simulink model "copia 15_10_26"  (R2026a)
settings: Solver=VariableStepAuto  StopTime=10  RelTol=1e-2  AbsTol=1e-2  EnableMultiTasking=on
values from neighbouring files (symbols this model uses):
  effective_bulkmodulus = 750e6    (= 750000000)    [MARLUP_hydr_params.m]
  m_load = 20    [MARLUP_hydr_params.m]
  p_supply = 160e5    (= 16000000)    [MARLUP_hydr_params.m]
  p_tank = 1.01325e5    (= 101325)    [MARLUP_hydr_params.m]
undefined symbols (not defined in the file or in its folder): cyl, Kd_heave, Kd_pitch, Kd_roll, Ki_heave, Ki_pitch, Ki_roll, Kp_heave, Kp_pitch, Kp_roll, pipe, Tinv, Ts, valve, X, Y, Z
libraries: sm_lib x75, nesl_utility x14, slpidlib x6, simulink x3
(part 4 of 5)

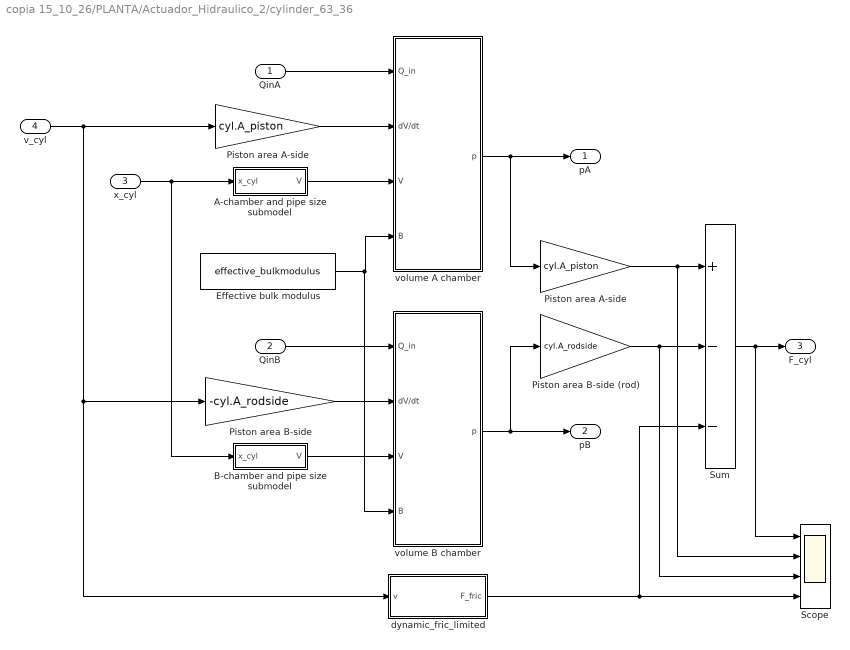
== system copia 15_10_26/PLANTA/Actuador_Hidraulico_2/cylinder_63_36 ==
  QinA : Inport
  QinB : Inport  Port=2
  x_cyl : Inport  Port=3
  v_cyl : Inport  Port=4
  A-chamber and pipe size submodel : Subsystem
  B-chamber and pipe size submodel : Subsystem
  Effective bulk modulus : Constant  Value=effective_bulkmodulus
  Piston area A-side : Gain  Gain=cyl.A_piston
  Piston area B-side (rod) : Gain  Gain=cyl.A_rodside
  Piston area A-side : Gain  Gain=cyl.A_piston
  Piston area B-side : Gain  Gain=-cyl.A_rodside
  Scope : Scope  NumInputPorts=4
      settings: ActiveDisplayYMinimum=-3356.48237  ActiveDisplayYMaximum=15799.75819
  Sum : Sum  Inputs=+--
  dynamic_fric_limited : Subsystem
  volume A chamber : Subsystem
  volume B chamber : Subsystem
  pA : Outport  VectorParamsAs1DForOutWhenUnconnected=off
  pB : Outport  Port=2  VectorParamsAs1DForOutWhenUnconnected=off
  F_cyl : Outport  Port=3  VectorParamsAs1DForOutWhenUnconnected=off
  wires:
  Piston area A-side/1 -> Scope/2, Sum/1
  volume A chamber/1(p) -> pA/1, Piston area A-side/1
  x_cyl/1 -> B-chamber and pipe size submodel/1(x_cyl), A-chamber and pipe size submodel/1(x_cyl)
  v_cyl/1 -> dynamic_fric_limited/1(v), Piston area B-side/1, Piston area A-side/1
  Piston area A-side/1 -> volume A chamber/2(" dV/dt")
  Effective bulk modulus/1 -> volume B chamber/4(" B"), volume A chamber/4(" B")
  Sum/1 -> Scope/1, F_cyl/1
  QinA/1 -> volume A chamber/1(Q_in)
  volume B chamber/1(p) -> pB/1, Piston area B-side (rod)/1
  Piston area B-side (rod)/1 -> Scope/3, Sum/2
  A-chamber and pipe size submodel/1(V) -> volume A chamber/3(" V")
  QinB/1 -> volume B chamber/1(Q_in)
  B-chamber and pipe size submodel/1(V) -> volume B chamber/3(" V")
  Piston area B-side/1 -> volume B chamber/2(" dV/dt")
  dynamic_fric_limited/1(F_fric) -> Sum/3, Scope/4

== system copia 15_10_26/PLANTA/Actuador_Hidraulico_2/gate_load_mass ==
  F_cyl : Inport
  Add : Sum
  Gain : Gain  Gain=1/m_load
  Integrator : Integrator
  Integrator1 : Integrator  InitialCondition=cyl.x_init
  load_fric : Subsystem
  x_cyl : Outport  VectorParamsAs1DForOutWhenUnconnected=off
  v_cyl : Outport  Port=2  VectorParamsAs1DForOutWhenUnconnected=off
  wires:
  Add/1 -> Gain/1
  Gain/1 -> Integrator/1  "accel"
  Integrator/1 -> load_fric/1(v), v_cyl/1, Integrator1/1  "velocity"
  Integrator1/1 -> x_cyl/1  "position"
  F_cyl/1 -> Add/1
  load_fric/1(F_fric_load) -> Add/2

== system copia 15_10_26/PLANTA/Actuador_Hidraulico_3/4_3_directional_valve ==
  pA : Inport
  pB : Inport  Port=2
  u : Inport  Port=3
  Port flows : Subsystem
  Relative opening of flow paths : Subsystem
  Supply pressure : Constant  Value=p_supply
  Tank pressure : Constant  Value=p_tank
  Valve dynamics : Subsystem
  QA : Outport  VectorParamsAs1DForOutWhenUnconnected=off
  QB : Outport  Port=2  VectorParamsAs1DForOutWhenUnconnected=off
  "Q_tank " : Outport  Port=3  VectorParamsAs1DForOutWhenUnconnected=off
  Q_pump : Outport  Port=4  VectorParamsAs1DForOutWhenUnconnected=off
  wires:
  pA/1 -> Port flows/5(pA)
  pB/1 -> Port flows/6(pB)
  Valve dynamics/1(x) -> Relative opening of flow paths/1(x)
  Port flows/3(Q from port T) -> "Q_tank "/1
  Port flows/4(Q from port S) -> Q_pump/1
  Relative opening of flow paths/1(av_SA) -> Port flows/1(av_SA)
  Relative opening of flow paths/2(av_AT) -> Port flows/2(av_AT)
  Relative opening of flow paths/4(av_SB) -> Port flows/4(av_SB)
  u/1 -> Valve dynamics/1(u)
  Port flows/2(Q from port A) -> QA/1
  Port flows/1(Q from port B) -> QB/1
  Supply pressure/1 -> Port flows/7(pS)
  Tank pressure/1 -> Port flows/8(pT)
  Relative opening of flow paths/3(av_BT) -> Port flows/3(av_BT)

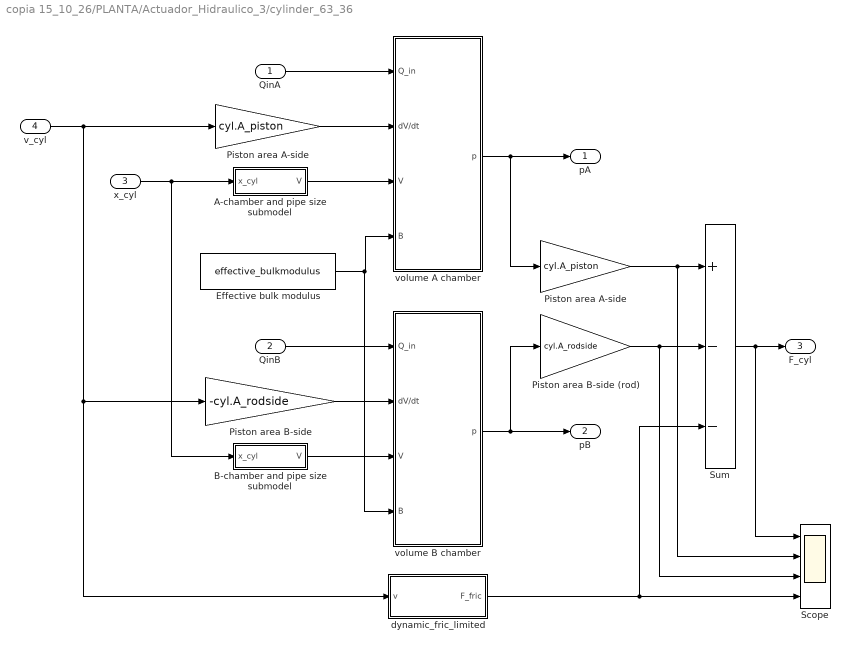
== system copia 15_10_26/PLANTA/Actuador_Hidraulico_3/cylinder_63_36 ==
  QinA : Inport
  QinB : Inport  Port=2
  x_cyl : Inport  Port=3
  v_cyl : Inport  Port=4
  A-chamber and pipe size submodel : Subsystem
  B-chamber and pipe size submodel : Subsystem
  Effective bulk modulus : Constant  Value=effective_bulkmodulus
  Piston area A-side : Gain  Gain=cyl.A_piston
  Piston area B-side (rod) : Gain  Gain=cyl.A_rodside
  Piston area A-side : Gain  Gain=cyl.A_piston
  Piston area B-side : Gain  Gain=-cyl.A_rodside
  Scope : Scope  NumInputPorts=4
      settings: ActiveDisplayYMinimum=-3356.48237  ActiveDisplayYMaximum=15799.75819
  Sum : Sum  Inputs=+--
  dynamic_fric_limited : Subsystem
  volume A chamber : Subsystem
  volume B chamber : Subsystem
  pA : Outport  VectorParamsAs1DForOutWhenUnconnected=off
  pB : Outport  Port=2  VectorParamsAs1DForOutWhenUnconnected=off
  F_cyl : Outport  Port=3  VectorParamsAs1DForOutWhenUnconnected=off
  wires:
  Piston area A-side/1 -> Scope/2, Sum/1
  volume A chamber/1(p) -> pA/1, Piston area A-side/1
  x_cyl/1 -> B-chamber and pipe size submodel/1(x_cyl), A-chamber and pipe size submodel/1(x_cyl)
  v_cyl/1 -> dynamic_fric_limited/1(v), Piston area B-side/1, Piston area A-side/1
  Piston area A-side/1 -> volume A chamber/2(" dV/dt")
  Effective bulk modulus/1 -> volume B chamber/4(" B"), volume A chamber/4(" B")
  Sum/1 -> Scope/1, F_cyl/1
  QinA/1 -> volume A chamber/1(Q_in)
  volume B chamber/1(p) -> pB/1, Piston area B-side (rod)/1
  Piston area B-side (rod)/1 -> Scope/3, Sum/2
  A-chamber and pipe size submodel/1(V) -> volume A chamber/3(" V")
  QinB/1 -> volume B chamber/1(Q_in)
  B-chamber and pipe size submodel/1(V) -> volume B chamber/3(" V")
  Piston area B-side/1 -> volume B chamber/2(" dV/dt")
  dynamic_fric_limited/1(F_fric) -> Sum/3, Scope/4

== system copia 15_10_26/PLANTA/Actuador_Hidraulico_3/gate_load_mass ==
  F_cyl : Inport
  Add : Sum
  Gain : Gain  Gain=1/m_load
  Integrator : Integrator
  Integrator1 : Integrator  InitialCondition=cyl.x_init
  load_fric : Subsystem
  x_cyl : Outport  VectorParamsAs1DForOutWhenUnconnected=off
  v_cyl : Outport  Port=2  VectorParamsAs1DForOutWhenUnconnected=off
  wires:
  Add/1 -> Gain/1
  Gain/1 -> Integrator/1  "accel"
  Integrator/1 -> load_fric/1(v), v_cyl/1, Integrator1/1  "velocity"
  Integrator1/1 -> x_cyl/1  "position"
  F_cyl/1 -> Add/1
  load_fric/1(F_fric_load) -> Add/2

== system copia 15_10_26/PLANTA/Piston 2/Garra 3 ==
  File Solid3 : sm_lib/Body Elements/File Solid  ExtGeomFileName=rotate.SLDPRT  UnitType=FromFile  ExtGeomFileUnits=m  StepReaderType=HEX  ExportConvexHullGeometry=off  InertiaType=CalculateFromGeometry  BasedOnType=DensityFromFile  Density=1000  DensityUnits=kg/m^3  Mass=1  MassUnits=kg  CenterOfMass=[0 0 0]  CenterOfMassUnits=m  MomentsOfInertia=[1 1 1]  MomentsOfInertiaUnits=kg*m^2  ProductsOfInertia=[0 0 0]  ProductsOfInertiaUnits=kg*m^2  GraphicType=FromGeometry  MarkerShape=Sphere  MarkerSize=10  GraphicVisPropType=SimpleVisualProperties  GraphicDiffuseColor=[0.5 0.5 0.5]  GraphicOpacity=1  GraphicSpecularColor=[0.5 0.5 0.5 1.0]  GraphicAmbientColor=[0.15 0.15 0.15 1.0]  GraphicEmissiveColor=[0.0 0.0 0.0 1.0]  GraphicShininess=75  DoExposeReferenceFrame=off  SerializedFrames=<Frames><Frame><Id>Frame2</Id><Value><Name>F2</Name><Origin><Source>GeometricFeature</Source><FeatureName>circular curve 40</FeatureName></Origin><PrimaryAxis><DefinedDirection>+Z</DefinedDirection><Source>ReferenceFrame</Source><SourceDirection>+Z</SourceDirection><FeatureName></FeatureName></PrimaryAxis><SecondaryAxis><DefinedDirection>+X</DefinedDirection><Source>ReferenceFrame</Source><SourceDirection>+X</SourceDirection><FeatureName></FeatureName></SecondaryAxis></Value></Frame><Frame><Id>Frame3</Id><Value><Name>F3-1</Name><Origin><Source>GeometricFeature</Source><FeatureName>planar surface 7</FeatureName></Origin><PrimaryAxis><DefinedDirection>+Z</DefinedDirection><Source>ReferenceFrame</Source><SourceDirection>+Z</SourceDirection><FeatureName></FeatureName></PrimaryAxis><SecondaryAxis><DefinedDirection>+X</DefinedDirection><Source>ReferenceFrame</Source><SourceDirection>+X</SourceDirection><FeatureName></FeatureName></SecondaryAxis></Value></Frame></Frames>
  Join block 1 : sm_lib/Body Elements/File Solid  ExtGeomFileName=joint_block.SLDPRT  UnitType=FromFile  ExtGeomFileUnits=m  StepReaderType=HEX  ExportConvexHullGeometry=off  InertiaType=CalculateFromGeometry  BasedOnType=DensityFromFile  Density=1000  DensityUnits=kg/m^3  Mass=1  MassUnits=kg  CenterOfMass=[0 0 0]  CenterOfMassUnits=m  MomentsOfInertia=[1 1 1]  MomentsOfInertiaUnits=kg*m^2  ProductsOfInertia=[0 0 0]  ProductsOfInertiaUnits=kg*m^2  GraphicType=FromGeometry  MarkerShape=Sphere  MarkerSize=10  GraphicVisPropType=SimpleVisualProperties  GraphicDiffuseColor=[0.5 0.5 0.5]  GraphicOpacity=1  GraphicSpecularColor=[0.5 0.5 0.5 1.0]  GraphicAmbientColor=[0.15 0.15 0.15 1.0]  GraphicEmissiveColor=[0.0 0.0 0.0 1.0]  GraphicShininess=75  DoExposeReferenceFrame=off  SerializedFrames=<Frames><Frame><Id>Frame1</Id><Value><Name>F1</Name><Origin><Source>GeometricFeature</Source><FeatureName>circular curve 40</FeatureName></Origin><PrimaryAxis><DefinedDirection>+Z</DefinedDirection><Source>ReferenceFrame</Source><SourceDirection>+X</SourceDirection><FeatureName></FeatureName></PrimaryAxis><SecondaryAxis><DefinedDirection>-X</DefinedDirection><Source>ReferenceFrame</Source><SourceDirection>+Z</SourceDirection><FeatureName></FeatureName></SecondaryAxis></Value></Frame><Frame><Id>Frame2</Id><Value><Name>F2</Name><Origin><Source>GeometricFeature</Source><FeatureName>circular curve 35</FeatureName></Origin><PrimaryAxis><DefinedDirection>+Z</DefinedDirection><Source>ReferenceFrame</Source><SourceDirection>+Z</SourceDirection><FeatureName></FeatureName></PrimaryAxis><SecondaryAxis><DefinedDirection>+X</DefinedDirection><Source>ReferenceFrame</Source><SourceDirection>+X</SourceDirection><FeatureName></FeatureName></SecondaryAxis></Value></Frame></Frames>
  Revolute Joint : sm_lib/Joints/Revolute Joint  JointMode=Normal  CompositeWrenchDir=FollowerOnBase  CompositeWrenchFrame=BaseFrame  SenseConstraintForce=off  SenseConstraintTorque=off  SenseTotalForce=off  SenseTotalTorque=off  PositionTargetSpecify=off  PositionTargetPriority=High  PositionTargetValue=-43.6009  PositionTargetValueUnits=deg  VelocityTargetSpecify=off  VelocityTargetPriority=High  VelocityTargetValue=0  VelocityTargetValueUnits=deg/s  EquilibriumPosition=0  EquilibriumPositionUnits=deg  SpringStiffness=0  SpringStiffnessUnits=N*m/deg  DampingCoefficient=1.5e-4  DampingCoefficientUnits=N*m/(deg/s)  LowerLimitSpecify=off  LowerLimitBound=-90  LowerLimitBoundUnits=deg  LowerLimitStiffness=1e4  LowerLimitStiffnessUnits=N*m/deg  LowerLimitDamping=10  LowerLimitDampingUnits=N*m/(deg/s)  LowerLimitTransitionRegionWidth=0.1  LowerLimitTransitionRegionWidthUnits=deg  UpperLimitSpecify=off  UpperLimitBound=90  UpperLimitBoundUnits=deg  UpperLimitStiffness=1e4  UpperLimitStiffnessUnits=N*m/deg  UpperLimitDamping=10  UpperLimitDampingUnits=N*m/(deg/s)  UpperLimitTransitionRegionWidth=0.1  UpperLimitTransitionRegionWidthUnits=deg  TorqueActuationMode=NoTorque  MotionActuationMode=ComputedMotion  SensePosition=off  SenseVelocity=off  SenseAcceleration=off  SenseTorqueForce=off  SenseLowerLimitTorqueForce=off  SenseUpperLimitTorqueForce=off
  Rigid Transform3 : sm_lib/Frames and Transforms/Rigid Transform  RotationMethod=RotationSequence  FollAlignAxisA=+X  BaseAlignAxisA=+Y  FollAlignAxisB=+Y  BaseAlignAxisB=+Z  RotationStandardAxis=+Y  RotationAngle=-30  RotationAngleUnits=deg  RotationArbitraryAxis=[0 0 1]  RotationSequenceAxes=FollowerAxes  RotationSequence=XYZ  RotationSequenceAngles=[2 -180 180]  RotationSequenceAnglesUnits=deg  RotationMatrix=[1 0 0;0 1 0;0 0 1]  Quaternion=[1 0 0 0]  TranslationMethod=None  TranslationCartesianOffset=[0 0 0]  TranslationCartesianOffsetUnits=m  TranslationStandardAxis=+Z  TranslationStandardOffset=0  TranslationStandardOffsetUnits=m  TranslationROffset=0  TranslationROffsetUnits=m  TranslationThetaOffset=0  TranslationThetaOffsetUnits=deg  TranslationZOffset=0  TranslationZOffsetUnits=m
  Rotate 1 : sm_lib/Body Elements/File Solid  ExtGeomFileName=rotate2.SLDPRT  UnitType=FromFile  ExtGeomFileUnits=m  StepReaderType=HEX  ExportConvexHullGeometry=off  InertiaType=CalculateFromGeometry  BasedOnType=DensityFromFile  Density=1000  DensityUnits=kg/m^3  Mass=1  MassUnits=kg  CenterOfMass=[0 0 0]  CenterOfMassUnits=m  MomentsOfInertia=[1 1 1]  MomentsOfInertiaUnits=kg*m^2  ProductsOfInertia=[0 0 0]  ProductsOfInertiaUnits=kg*m^2  GraphicType=FromGeometry  MarkerShape=Sphere  MarkerSize=10  GraphicVisPropType=SimpleVisualProperties  GraphicDiffuseColor=[0.5 0.5 0.5]  GraphicOpacity=1  GraphicSpecularColor=[0.5 0.5 0.5 1.0]  GraphicAmbientColor=[0.15 0.15 0.15 1.0]  GraphicEmissiveColor=[0.0 0.0 0.0 1.0]  GraphicShininess=75  DoExposeReferenceFrame=off  SerializedFrames=<Frames><Frame><Id>Frame1</Id><Value><Name>F1</Name><Origin><Source>GeometricFeature</Source><FeatureName>circular curve 36</FeatureName></Origin><PrimaryAxis><DefinedDirection>+Y</DefinedDirection><Source>ReferenceFrame</Source><SourceDirection>+Z</SourceDirection><FeatureName></FeatureName></PrimaryAxis><SecondaryAxis><DefinedDirection>+X</DefinedDirection><Source>ReferenceFrame</Source><SourceDirection>+X</SourceDirection><FeatureName></FeatureName></SecondaryAxis></Value></Frame><Frame><Id>Frame2</Id><Value><Name>F2</Name><Origin><Source>GeometricFeature</Source><FeatureName>circular curve 43</FeatureName></Origin><PrimaryAxis><DefinedDirection>+Z</DefinedDirection><Source>ReferenceFrame</Source><SourceDirection>+X</SourceDirection><FeatureName></FeatureName></PrimaryAxis><SecondaryAxis><DefinedDirection>-X</DefinedDirection><Source>ReferenceFrame</Source><SourceDirection>+Z</SourceDirection><FeatureName></FeatureName></SecondaryAxis></Value></Frame></Frames>
  Conn1 : PMIOPort  Side=Left
  Conn2 : PMIOPort  Port=2  Side=Right
  measure_up : PMIOPort  Port=3  Side=Right
  measure_z : PMIOPort  Port=4  Side=Left
  connections:
  Rigid Transform3/LConn1 -- measure_up/RConn1 -- Join block 1/RConn1
  Rotate 1/LConn1 -- Conn1/RConn1
  Conn2/RConn1 -- File Solid3/RConn1
  Rotate 1/RConn1 -- Revolute Joint/LConn1
  Join block 1/LConn1 -- measure_z/RConn1 -- Revolute Joint/RConn1
  File Solid3/LConn1 -- Rigid Transform3/RConn1

== system copia 15_10_26/PLANTA/Piston1/Garra 1 ==
  File Solid1 : sm_lib/Body Elements/File Solid  ExtGeomFileName=rotate.SLDPRT  UnitType=FromFile  ExtGeomFileUnits=m  StepReaderType=HEX  ExportConvexHullGeometry=off  InertiaType=CalculateFromGeometry  BasedOnType=DensityFromFile  Density=1000  DensityUnits=kg/m^3  Mass=1  MassUnits=kg  CenterOfMass=[0 0 0]  CenterOfMassUnits=m  MomentsOfInertia=[1 1 1]  MomentsOfInertiaUnits=kg*m^2  ProductsOfInertia=[0 0 0]  ProductsOfInertiaUnits=kg*m^2  GraphicType=FromGeometry  MarkerShape=Sphere  MarkerSize=10  GraphicVisPropType=SimpleVisualProperties  GraphicDiffuseColor=[0.5 0.5 0.5]  GraphicOpacity=1  GraphicSpecularColor=[0.5 0.5 0.5 1.0]  GraphicAmbientColor=[0.15 0.15 0.15 1.0]  GraphicEmissiveColor=[0.0 0.0 0.0 1.0]  GraphicShininess=75  DoExposeReferenceFrame=off  SerializedFrames=<Frames><Frame><Id>Frame2</Id><Value><Name>F2</Name><Origin><Source>GeometricFeature</Source><FeatureName>circular curve 40</FeatureName></Origin><PrimaryAxis><DefinedDirection>+Z</DefinedDirection><Source>ReferenceFrame</Source><SourceDirection>+Z</SourceDirection><FeatureName></FeatureName></PrimaryAxis><SecondaryAxis><DefinedDirection>+X</DefinedDirection><Source>ReferenceFrame</Source><SourceDirection>+X</SourceDirection><FeatureName></FeatureName></SecondaryAxis></Value></Frame><Frame><Id>Frame3</Id><Value><Name>F3-1</Name><Origin><Source>GeometricFeature</Source><FeatureName>planar surface 7</FeatureName></Origin><PrimaryAxis><DefinedDirection>+Z</DefinedDirection><Source>ReferenceFrame</Source><SourceDirection>+Z</SourceDirection><FeatureName></FeatureName></PrimaryAxis><SecondaryAxis><DefinedDirection>+X</DefinedDirection><Source>ReferenceFrame</Source><SourceDirection>+X</SourceDirection><FeatureName></FeatureName></SecondaryAxis></Value></Frame></Frames>
  Join block 2 : sm_lib/Body Elements/File Solid  ExtGeomFileName=joint_block.SLDPRT  UnitType=FromFile  ExtGeomFileUnits=m  StepReaderType=HEX  ExportConvexHullGeometry=off  InertiaType=CalculateFromGeometry  BasedOnType=DensityFromFile  Density=1000  DensityUnits=kg/m^3  Mass=1  MassUnits=kg  CenterOfMass=[0 0 0]  CenterOfMassUnits=m  MomentsOfInertia=[1 1 1]  MomentsOfInertiaUnits=kg*m^2  ProductsOfInertia=[0 0 0]  ProductsOfInertiaUnits=kg*m^2  GraphicType=FromGeometry  MarkerShape=Sphere  MarkerSize=10  GraphicVisPropType=SimpleVisualProperties  GraphicDiffuseColor=[0.5 0.5 0.5]  GraphicOpacity=1  GraphicSpecularColor=[0.5 0.5 0.5 1.0]  GraphicAmbientColor=[0.15 0.15 0.15 1.0]  GraphicEmissiveColor=[0.0 0.0 0.0 1.0]  GraphicShininess=75  DoExposeReferenceFrame=off  SerializedFrames=<Frames><Frame><Id>Frame1</Id><Value><Name>F1</Name><Origin><Source>GeometricFeature</Source><FeatureName>circular curve 40</FeatureName></Origin><PrimaryAxis><DefinedDirection>+Z</DefinedDirection><Source>ReferenceFrame</Source><SourceDirection>+X</SourceDirection><FeatureName></FeatureName></PrimaryAxis><SecondaryAxis><DefinedDirection>-X</DefinedDirection><Source>ReferenceFrame</Source><SourceDirection>+Z</SourceDirection><FeatureName></FeatureName></SecondaryAxis></Value></Frame><Frame><Id>Frame2</Id><Value><Name>F2</Name><Origin><Source>GeometricFeature</Source><FeatureName>circular curve 35</FeatureName></Origin><PrimaryAxis><DefinedDirection>+Z</DefinedDirection><Source>ReferenceFrame</Source><SourceDirection>+Z</SourceDirection><FeatureName></FeatureName></PrimaryAxis><SecondaryAxis><DefinedDirection>+X</DefinedDirection><Source>ReferenceFrame</Source><SourceDirection>+X</SourceDirection><FeatureName></FeatureName></SecondaryAxis></Value></Frame></Frames>
  Revolute Joint : sm_lib/Joints/Revolute Joint  JointMode=Normal  CompositeWrenchDir=FollowerOnBase  CompositeWrenchFrame=BaseFrame  SenseConstraintForce=off  SenseConstraintTorque=off  SenseTotalForce=off  SenseTotalTorque=off  PositionTargetSpecify=off  PositionTargetPriority=High  PositionTargetValue=-45.85  PositionTargetValueUnits=deg  VelocityTargetSpecify=off  VelocityTargetPriority=High  VelocityTargetValue=0  VelocityTargetValueUnits=deg/s  EquilibriumPosition=0  EquilibriumPositionUnits=deg  SpringStiffness=0  SpringStiffnessUnits=N*m/deg  DampingCoefficient=1.5e-4  DampingCoefficientUnits=N*m/(deg/s)  LowerLimitSpecify=off  LowerLimitBound=-90  LowerLimitBoundUnits=deg  LowerLimitStiffness=1e4  LowerLimitStiffnessUnits=N*m/deg  LowerLimitDamping=10  LowerLimitDampingUnits=N*m/(deg/s)  LowerLimitTransitionRegionWidth=0.1  LowerLimitTransitionRegionWidthUnits=deg  UpperLimitSpecify=off  UpperLimitBound=90  UpperLimitBoundUnits=deg  UpperLimitStiffness=1e4  UpperLimitStiffnessUnits=N*m/deg  UpperLimitDamping=10  UpperLimitDampingUnits=N*m/(deg/s)  UpperLimitTransitionRegionWidth=0.1  UpperLimitTransitionRegionWidthUnits=deg  TorqueActuationMode=NoTorque  MotionActuationMode=ComputedMotion  SensePosition=off  SenseVelocity=off  SenseAcceleration=off  SenseTorqueForce=off  SenseLowerLimitTorqueForce=off  SenseUpperLimitTorqueForce=off
  Rigid Transform3 : sm_lib/Frames and Transforms/Rigid Transform  RotationMethod=RotationSequence  FollAlignAxisA=+X  BaseAlignAxisA=+Y  FollAlignAxisB=+Y  BaseAlignAxisB=+Z  RotationStandardAxis=+Y  RotationAngle=-30  RotationAngleUnits=deg  RotationArbitraryAxis=[0 0 1]  RotationSequenceAxes=FollowerAxes  RotationSequence=XYZ  RotationSequenceAngles=[2 -180 180]  RotationSequenceAnglesUnits=deg  RotationMatrix=[1 0 0;0 1 0;0 0 1]  Quaternion=[1 0 0 0]  TranslationMethod=None  TranslationCartesianOffset=[0 0 0]  TranslationCartesianOffsetUnits=m  TranslationStandardAxis=+Z  TranslationStandardOffset=0  TranslationStandardOffsetUnits=m  TranslationROffset=0  TranslationROffsetUnits=m  TranslationThetaOffset=0  TranslationThetaOffsetUnits=deg  TranslationZOffset=0  TranslationZOffsetUnits=m
  Rotate 2 : sm_lib/Body Elements/File Solid  ExtGeomFileName=rotate2.SLDPRT  UnitType=FromFile  ExtGeomFileUnits=m  StepReaderType=HEX  ExportConvexHullGeometry=off  InertiaType=CalculateFromGeometry  BasedOnType=DensityFromFile  Density=1000  DensityUnits=kg/m^3  Mass=1  MassUnits=kg  CenterOfMass=[0 0 0]  CenterOfMassUnits=m  MomentsOfInertia=[1 1 1]  MomentsOfInertiaUnits=kg*m^2  ProductsOfInertia=[0 0 0]  ProductsOfInertiaUnits=kg*m^2  GraphicType=FromGeometry  MarkerShape=Sphere  MarkerSize=10  GraphicVisPropType=SimpleVisualProperties  GraphicDiffuseColor=[0.5 0.5 0.5]  GraphicOpacity=1  GraphicSpecularColor=[0.5 0.5 0.5 1.0]  GraphicAmbientColor=[0.15 0.15 0.15 1.0]  GraphicEmissiveColor=[0.0 0.0 0.0 1.0]  GraphicShininess=75  DoExposeReferenceFrame=off  SerializedFrames=<Frames><Frame><Id>Frame1</Id><Value><Name>F1</Name><Origin><Source>GeometricFeature</Source><FeatureName>circular curve 36</FeatureName></Origin><PrimaryAxis><DefinedDirection>+Y</DefinedDirection><Source>ReferenceFrame</Source><SourceDirection>+Z</SourceDirection><FeatureName></FeatureName></PrimaryAxis><SecondaryAxis><DefinedDirection>+X</DefinedDirection><Source>ReferenceFrame</Source><SourceDirection>+X</SourceDirection><FeatureName></FeatureName></SecondaryAxis></Value></Frame><Frame><Id>Frame2</Id><Value><Name>F2</Name><Origin><Source>GeometricFeature</Source><FeatureName>circular curve 43</FeatureName></Origin><PrimaryAxis><DefinedDirection>+Z</DefinedDirection><Source>ReferenceFrame</Source><SourceDirection>+X</SourceDirection><FeatureName></FeatureName></PrimaryAxis><SecondaryAxis><DefinedDirection>-X</DefinedDirection><Source>ReferenceFrame</Source><SourceDirection>+Z</SourceDirection><FeatureName></FeatureName></SecondaryAxis></Value></Frame></Frames>
  Conn1 : PMIOPort  Side=Left
  Conn2 : PMIOPort  Port=2  Side=Right
  connections:
  Rotate 2/LConn1 -- Conn1/RConn1
  File Solid1/RConn1 -- Conn2/RConn1
  Rigid Transform3/RConn1 -- File Solid1/LConn1
  Rotate 2/RConn1 -- Revolute Joint/LConn1
  Revolute Joint/RConn1 -- Join block 2/LConn1
  Join block 2/RConn1 -- Rigid Transform3/LConn1

== system copia 15_10_26/PLANTA/Piston3/Garra 3 ==
  File Solid3 : sm_lib/Body Elements/File Solid  ExtGeomFileName=rotate.SLDPRT  UnitType=FromFile  ExtGeomFileUnits=m  StepReaderType=HEX  ExportConvexHullGeometry=off  InertiaType=CalculateFromGeometry  BasedOnType=DensityFromFile  Density=1000  DensityUnits=kg/m^3  Mass=1  MassUnits=kg  CenterOfMass=[0 0 0]  CenterOfMassUnits=m  MomentsOfInertia=[1 1 1]  MomentsOfInertiaUnits=kg*m^2  ProductsOfInertia=[0 0 0]  ProductsOfInertiaUnits=kg*m^2  GraphicType=FromGeometry  MarkerShape=Sphere  MarkerSize=10  GraphicVisPropType=SimpleVisualProperties  GraphicDiffuseColor=[0.5 0.5 0.5]  GraphicOpacity=1  GraphicSpecularColor=[0.5 0.5 0.5 1.0]  GraphicAmbientColor=[0.15 0.15 0.15 1.0]  GraphicEmissiveColor=[0.0 0.0 0.0 1.0]  GraphicShininess=75  DoExposeReferenceFrame=off  SerializedFrames=<Frames><Frame><Id>Frame1</Id><Value><Name>F1</Name><Origin><Source>GeometricFeature</Source><FeatureName>circular curve 16</FeatureName></Origin><PrimaryAxis><DefinedDirection>+Z</DefinedDirection><Source>ReferenceFrame</Source><SourceDirection>+Z</SourceDirection><FeatureName></FeatureName></PrimaryAxis><SecondaryAxis><DefinedDirection>+X</DefinedDirection><Source>ReferenceFrame</Source><SourceDirection>+X</SourceDirection><FeatureName></FeatureName></SecondaryAxis></Value></Frame><Frame><Id>Frame2</Id><Value><Name>F2</Name><Origin><Source>GeometricFeature</Source><FeatureName>circular curve 40</FeatureName></Origin><PrimaryAxis><DefinedDirection>+Z</DefinedDirection><Source>ReferenceFrame</Source><SourceDirection>+Z</SourceDirection><FeatureName></FeatureName></PrimaryAxis><SecondaryAxis><DefinedDirection>+X</DefinedDirection><Source>ReferenceFrame</Source><SourceDirection>+X</SourceDirection><FeatureName></FeatureName></SecondaryAxis></Value></Frame><Frame><Id>Frame3</Id><Value><Name>F3-1</Name><Origin><Source>GeometricFeature</Source><FeatureName>planar surface 7</FeatureName></Origin><PrimaryAxis><DefinedDirection>+Z</DefinedDirection><Source>ReferenceFrame</Source><SourceDirection>+Z</SourceDirection><FeatureName></FeatureName></PrimaryAxis><SecondaryAxis><DefinedDirection>+X</DefinedDirection><Source>ReferenceFrame</Source><SourceDirection>+X</SourceDirection><FeatureName></FeatureName></SecondaryAxis></Value></Frame></Frames>
  Join block 1 : sm_lib/Body Elements/File Solid  ExtGeomFileName=joint_block.SLDPRT  UnitType=FromFile  ExtGeomFileUnits=m  StepReaderType=HEX  ExportConvexHullGeometry=off  InertiaType=CalculateFromGeometry  BasedOnType=DensityFromFile  Density=1000  DensityUnits=kg/m^3  Mass=1  MassUnits=kg  CenterOfMass=[0 0 0]  CenterOfMassUnits=m  MomentsOfInertia=[1 1 1]  MomentsOfInertiaUnits=kg*m^2  ProductsOfInertia=[0 0 0]  ProductsOfInertiaUnits=kg*m^2  GraphicType=FromGeometry  MarkerShape=Sphere  MarkerSize=10  GraphicVisPropType=SimpleVisualProperties  GraphicDiffuseColor=[0.5 0.5 0.5]  GraphicOpacity=1  GraphicSpecularColor=[0.5 0.5 0.5 1.0]  GraphicAmbientColor=[0.15 0.15 0.15 1.0]  GraphicEmissiveColor=[0.0 0.0 0.0 1.0]  GraphicShininess=75  DoExposeReferenceFrame=off  SerializedFrames=<Frames><Frame><Id>Frame1</Id><Value><Name>F1</Name><Origin><Source>GeometricFeature</Source><FeatureName>circular curve 40</FeatureName></Origin><PrimaryAxis><DefinedDirection>+Z</DefinedDirection><Source>ReferenceFrame</Source><SourceDirection>+X</SourceDirection><FeatureName></FeatureName></PrimaryAxis><SecondaryAxis><DefinedDirection>-X</DefinedDirection><Source>ReferenceFrame</Source><SourceDirection>+Z</SourceDirection><FeatureName></FeatureName></SecondaryAxis></Value></Frame><Frame><Id>Frame2</Id><Value><Name>F2</Name><Origin><Source>GeometricFeature</Source><FeatureName>circular curve 35</FeatureName></Origin><PrimaryAxis><DefinedDirection>+Z</DefinedDirection><Source>ReferenceFrame</Source><SourceDirection>+Z</SourceDirection><FeatureName></FeatureName></PrimaryAxis><SecondaryAxis><DefinedDirection>+X</DefinedDirection><Source>ReferenceFrame</Source><SourceDirection>+X</SourceDirection><FeatureName></FeatureName></SecondaryAxis></Value></Frame></Frames>
  Revolute Joint : sm_lib/Joints/Revolute Joint  JointMode=Normal  CompositeWrenchDir=FollowerOnBase  CompositeWrenchFrame=BaseFrame  SenseConstraintForce=off  SenseConstraintTorque=off  SenseTotalForce=off  SenseTotalTorque=off  PositionTargetSpecify=off  PositionTargetPriority=High  PositionTargetValue=-43.492  PositionTargetValueUnits=deg  VelocityTargetSpecify=off  VelocityTargetPriority=High  VelocityTargetValue=0  VelocityTargetValueUnits=deg/s  EquilibriumPosition=0  EquilibriumPositionUnits=deg  SpringStiffness=0  SpringStiffnessUnits=N*m/deg  DampingCoefficient=1.5e-4  DampingCoefficientUnits=N*m/(deg/s)  LowerLimitSpecify=off  LowerLimitBound=-90  LowerLimitBoundUnits=deg  LowerLimitStiffness=1e4  LowerLimitStiffnessUnits=N*m/deg  LowerLimitDamping=10  LowerLimitDampingUnits=N*m/(deg/s)  LowerLimitTransitionRegionWidth=0.1  LowerLimitTransitionRegionWidthUnits=deg  UpperLimitSpecify=off  UpperLimitBound=90  UpperLimitBoundUnits=deg  UpperLimitStiffness=1e4  UpperLimitStiffnessUnits=N*m/deg  UpperLimitDamping=10  UpperLimitDampingUnits=N*m/(deg/s)  UpperLimitTransitionRegionWidth=0.1  UpperLimitTransitionRegionWidthUnits=deg  TorqueActuationMode=NoTorque  MotionActuationMode=ComputedMotion  SensePosition=off  SenseVelocity=off  SenseAcceleration=off  SenseTorqueForce=off  SenseLowerLimitTorqueForce=off  SenseUpperLimitTorqueForce=off
  Rigid Transform3 : sm_lib/Frames and Transforms/Rigid Transform  RotationMethod=RotationSequence  FollAlignAxisA=+X  BaseAlignAxisA=+Y  FollAlignAxisB=+Y  BaseAlignAxisB=+Z  RotationStandardAxis=+Y  RotationAngle=-30  RotationAngleUnits=deg  RotationArbitraryAxis=[0 0 1]  RotationSequenceAxes=FollowerAxes  RotationSequence=XYZ  RotationSequenceAngles=[2 -180 180]  RotationSequenceAnglesUnits=deg  RotationMatrix=[1 0 0;0 1 0;0 0 1]  Quaternion=[1 0 0 0]  TranslationMethod=None  TranslationCartesianOffset=[0 0 0]  TranslationCartesianOffsetUnits=m  TranslationStandardAxis=+Z  TranslationStandardOffset=0  TranslationStandardOffsetUnits=m  TranslationROffset=0  TranslationROffsetUnits=m  TranslationThetaOffset=0  TranslationThetaOffsetUnits=deg  TranslationZOffset=0  TranslationZOffsetUnits=m
  Rotate 1 : sm_lib/Body Elements/File Solid  ExtGeomFileName=rotate2.SLDPRT  UnitType=FromFile  ExtGeomFileUnits=m  StepReaderType=HEX  ExportConvexHullGeometry=off  InertiaType=CalculateFromGeometry  BasedOnType=DensityFromFile  Density=1000  DensityUnits=kg/m^3  Mass=1  MassUnits=kg  CenterOfMass=[0 0 0]  CenterOfMassUnits=m  MomentsOfInertia=[1 1 1]  MomentsOfInertiaUnits=kg*m^2  ProductsOfInertia=[0 0 0]  ProductsOfInertiaUnits=kg*m^2  GraphicType=FromGeometry  MarkerShape=Sphere  MarkerSize=10  GraphicVisPropType=SimpleVisualProperties  GraphicDiffuseColor=[0.5 0.5 0.5]  GraphicOpacity=1  GraphicSpecularColor=[0.5 0.5 0.5 1.0]  GraphicAmbientColor=[0.15 0.15 0.15 1.0]  GraphicEmissiveColor=[0.0 0.0 0.0 1.0]  GraphicShininess=75  DoExposeReferenceFrame=off  SerializedFrames=<Frames><Frame><Id>Frame1</Id><Value><Name>F1</Name><Origin><Source>GeometricFeature</Source><FeatureName>circular curve 36</FeatureName></Origin><PrimaryAxis><DefinedDirection>+Y</DefinedDirection><Source>ReferenceFrame</Source><SourceDirection>+Z</SourceDirection><FeatureName></FeatureName></PrimaryAxis><SecondaryAxis><DefinedDirection>+X</DefinedDirection><Source>ReferenceFrame</Source><SourceDirection>+X</SourceDirection><FeatureName></FeatureName></SecondaryAxis></Value></Frame><Frame><Id>Frame2</Id><Value><Name>F2</Name><Origin><Source>GeometricFeature</Source><FeatureName>circular curve 43</FeatureName></Origin><PrimaryAxis><DefinedDirection>+Z</DefinedDirection><Source>ReferenceFrame</Source><SourceDirection>+X</SourceDirection><FeatureName></FeatureName></PrimaryAxis><SecondaryAxis><DefinedDirection>-X</DefinedDirection><Source>ReferenceFrame</Source><SourceDirection>+Z</SourceDirection><FeatureName></FeatureName></SecondaryAxis></Value></Frame></Frames>
  Conn1 : PMIOPort  Side=Left
  Conn2 : PMIOPort  Port=2  Side=Right
  connections:
  Join block 1/RConn1 -- Rigid Transform3/LConn1
  Rigid Transform3/RConn1 -- File Solid3/RConn1
  Rotate 1/LConn1 -- Conn1/RConn1
  File Solid3/LConn2 -- Conn2/RConn1
  Rotate 1/RConn1 -- Revolute Joint/LConn1
  Join block 1/LConn1 -- Revolute Joint/RConn1

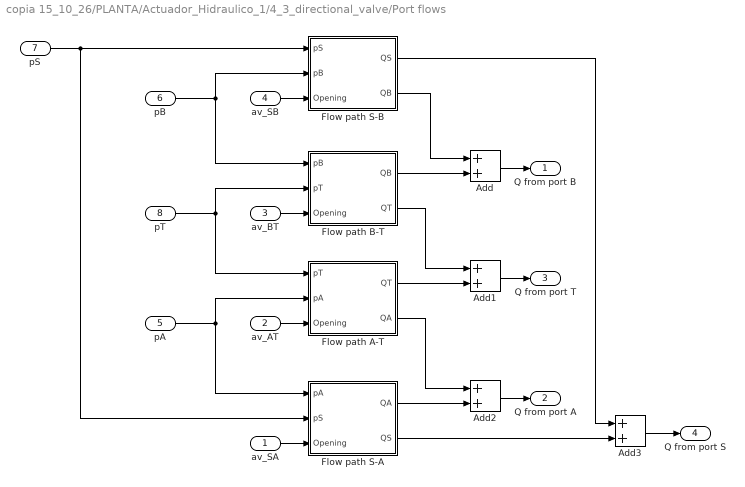
== system copia 15_10_26/PLANTA/Actuador_Hidraulico_1/4_3_directional_valve/Port flows ==
  av_SA : Inport
  av_AT : Inport  Port=2
  av_BT : Inport  Port=3
  av_SB : Inport  Port=4
  pA : Inport  Port=5
  pB : Inport  Port=6
  pS : Inport  Port=7
  pT : Inport  Port=8
  Add{,1..3} (4 alike) : Sum
  Flow path A-T : Subsystem  mask(Hydraulic){DPN=valve.dpN, QN=valve.QN, ptr=valve.ptr}
      mask prompts: DPN "Nominal Pressure Difference [Pa] :"; QN "Flow at nominal pressure difference and maximum opening [m^3/s] :"; ptr "Transition pressure [Pa] :"
      mask help:
      | Implements numerically robust turbulent flow equation. Polynomial flow equation is
      | used when abs(dp) is smaller than transition pressure.
      | [Source: Ellman, A. & Piche, R. 1996.
      | A Modified Orifice Flow Formula for Numerical Simulation of Fluid Power Systems.
      | Fluid Power Systems and Technology, ASME]
      mask init:
      | K = QN/(sqrt(DPN));
  Flow path B-T : Subsystem  mask(Hydraulic){DPN=valve.dpN, QN=valve.QN, ptr=valve.ptr}
      mask prompts: DPN "Nominal Pressure Difference [Pa] :"; QN "Flow at nominal pressure difference and maximum opening [m^3/s] :"; ptr "Transition pressure [Pa] :"
      mask help:
      | Implements numerically robust turbulent flow equation. Polynomial flow equation is
      | used when abs(dp) is smaller than transition pressure.
      | [Source: Ellman, A. & Piche, R. 1996.
      | A Modified Orifice Flow Formula for Numerical Simulation of Fluid Power Systems.
      | Fluid Power Systems and Technology, ASME]
      mask init:
      | K = QN/(sqrt(DPN));
  Flow path S-A : Subsystem  mask(Hydraulic){DPN=valve.dpN, QN=valve.QN, ptr=valve.ptr}
      mask prompts: DPN "Nominal Pressure Difference [Pa] :"; QN "Flow at nominal pressure difference and maximum opening [m^3/s] :"; ptr "Transition pressure [Pa] :"
      mask help:
      | Implements numerically robust turbulent flow equation. Polynomial flow equation is
      | used when abs(dp) is smaller than transition pressure.
      | [Source: Ellman, A. & Piche, R. 1996.
      | A Modified Orifice Flow Formula for Numerical Simulation of Fluid Power Systems.
      | Fluid Power Systems and Technology, ASME]
      mask init:
      | K = QN/(sqrt(DPN));
  Flow path S-B : Subsystem  mask(Hydraulic){DPN=valve.dpN, QN=valve.QN, ptr=valve.ptr}
      mask prompts: DPN "Nominal Pressure Difference [Pa] :"; QN "Flow at nominal pressure difference and maximum opening [m^3/s] :"; ptr "Transition pressure [Pa] :"
      mask help:
      | Implements numerically robust turbulent flow equation. Polynomial flow equation is
      | used when abs(dp) is smaller than transition pressure.
      | [Source: Ellman, A. & Piche, R. 1996.
      | A Modified Orifice Flow Formula for Numerical Simulation of Fluid Power Systems.
      | Fluid Power Systems and Technology, ASME]
      mask init:
      | K = QN/(sqrt(DPN));
  Q from port B : Outport  VectorParamsAs1DForOutWhenUnconnected=off
  Q from port A : Outport  Port=2  VectorParamsAs1DForOutWhenUnconnected=off
  Q from port T : Outport  Port=3  VectorParamsAs1DForOutWhenUnconnected=off
  Q from port S : Outport  Port=4  VectorParamsAs1DForOutWhenUnconnected=off
  wires:
  av_SA/1 -> Flow path S-A/3(Opening)
  av_AT/1 -> Flow path A-T/3(Opening)
  av_BT/1 -> Flow path B-T/3(Opening)
  pA/1 -> Flow path A-T/2(pA), Flow path S-A/1(pA)
  pB/1 -> Flow path B-T/1(pB), Flow path S-B/2(pB)
  pS/1 -> Flow path S-B/1(pS), Flow path S-A/2(pS)
  pT/1 -> Flow path A-T/1(pT), Flow path B-T/2(pT)
  Add/1 -> Q from port B/1
  Add1/1 -> Q from port T/1
  Add2/1 -> Q from port A/1
  Add3/1 -> Q from port S/1
  Flow path S-B/1(QS) -> Add3/1
  Flow path S-A/2(QS) -> Add3/2
  Flow path S-A/1(QA) -> Add2/2
  Flow path A-T/2(QA) -> Add2/1
  Flow path A-T/1(QT) -> Add1/2
  Flow path B-T/2(QT) -> Add1/1
  Flow path B-T/1(QB) -> Add/2
  Flow path S-B/2(QB) -> Add/1
  av_SB/1 -> Flow path S-B/3(Opening)

== system copia 15_10_26/PLANTA/Actuador_Hidraulico_1/4_3_directional_valve/Relative opening of flow paths ==
  x : Inport
  Gain : Gain  Gain=-1
  Lookup Table5 : Lookup  InputValues=[0.01 0.05 0.1 0.2 0.3 0.4 1]  Table=[0.01 0.039 0.078 0.16 0.23 0.31 0.78]  SaturateOnIntegerOverflow=off
  Lookup Table6 : Lookup  InputValues=[0.01 0.05 0.1 0.2 0.3 0.4 1]  Table=[0.01 0.036 0.072 0.14 0.22 0.29 0.72]  SaturateOnIntegerOverflow=off
  Lookup Table7 : Lookup  InputValues=[0.01 0.05 0.1 0.2 0.3 0.4 1]  Table=[0.01 0.039 0.077 0.15 0.23 0.31 0.77]  SaturateOnIntegerOverflow=off
  Lookup Table8 : Lookup  InputValues=[0.01 0.05 0.1 0.2 0.3 0.4 1]  Table=[0.01 0.035 0.070 0.14 0.21 0.28 0.70]  SaturateOnIntegerOverflow=off
  Saturation1 : Saturate  UpperLimit=1  LowerLimit=0
  Saturation2 : Saturate  UpperLimit=0  LowerLimit=-1
  av_SA : Outport  VectorParamsAs1DForOutWhenUnconnected=off
  av_AT : Outport  Port=2  VectorParamsAs1DForOutWhenUnconnected=off
  av_BT : Outport  Port=3  VectorParamsAs1DForOutWhenUnconnected=off
  av_SB : Outport  Port=4  VectorParamsAs1DForOutWhenUnconnected=off
  wires:
  x/1 -> Saturation2/1, Saturation1/1
  Saturation2/1 -> Gain/1
  Lookup Table8/1 -> av_AT/1
  Lookup Table7/1 -> av_SB/1
  Lookup Table6/1 -> av_BT/1
  Lookup Table5/1 -> av_SA/1
  Saturation1/1 -> Lookup Table5/1, Lookup Table6/1
  Gain/1 -> Lookup Table8/1, Lookup Table7/1

== system copia 15_10_26/PLANTA/Actuador_Hidraulico_1/4_3_directional_valve/Valve dynamics ==
  u : Inport
  Rate Limiter : RateLimiter  RisingSlewLimit=valve.ratelimit  FallingSlewLimit=-valve.ratelimit  SampleTimeMode=inherited
  Saturation limits [-1,1] : Saturate  UpperLimit=1  LowerLimit=-1
  Saturation limits [-1,1]2 : Saturate  UpperLimit=1  LowerLimit=-1
  Transfer Fcn1 : TransferFcn  Denominator=[valve.tau 1]
  Transport Delay of the valve : TransportDelay  DelayTime=valve.delay
  x : Outport  VectorParamsAs1DForOutWhenUnconnected=off
  wires:
  Saturation limits [-1,1]/1 -> Transport Delay of the valve/1
  Transport Delay of the valve/1 -> Rate Limiter/1
  Rate Limiter/1 -> Transfer Fcn1/1
  u/1 -> Saturation limits [-1,1]/1
  Transfer Fcn1/1 -> Saturation limits [-1,1]2/1
  Saturation limits [-1,1]2/1 -> x/1

== system copia 15_10_26/PLANTA/Actuador_Hidraulico_1/cylinder_63_36/A-chamber and pipe size submodel ==
  x_cyl : Inport
  A : Gain  Gain=pipe.area
  A chamber dead volume : Constant  Value=cyl.V0A
  Add : Sum  Inputs=+++
  Gain : Gain  Gain=cyl.A_piston
  Lenght : Constant  Value=pipe.lenght
  V : Outport  VectorParamsAs1DForOutWhenUnconnected=off
  wires:
  A/1 -> Add/3
  Lenght/1 -> A/1
  A chamber dead volume/1 -> Add/2
  Gain/1 -> Add/1
  x_cyl/1 -> Gain/1
  Add/1 -> V/1

== system copia 15_10_26/PLANTA/Actuador_Hidraulico_1/cylinder_63_36/B-chamber and pipe size submodel ==
  x_cyl : Inport
  A : Gain  Gain=pipe.area
  Add : Sum  Inputs=+-
  Add1 : Sum  Inputs=+++
  B chamber dead volume : Constant  Value=cyl.V0B
  Cylinder stroke : Constant  Value=cyl.stroke
  Gain1 : Gain  Gain=cyl.A_rodside
  Lenght : Constant  Value=pipe.lenght
  V : Outport  VectorParamsAs1DForOutWhenUnconnected=off
  wires:
  A/1 -> Add1/3
  Lenght/1 -> A/1
  Cylinder stroke/1 -> Add/1
  Gain1/1 -> Add1/1
  Add/1 -> Gain1/1
  x_cyl/1 -> Add/2
  B chamber dead volume/1 -> Add1/2
  Add1/1 -> V/1

== system copia 15_10_26/PLANTA/Actuador_Hidraulico_1/cylinder_63_36/dynamic_fric_limited ==
  v : Inport
  Abs : Abs  SaturateOnIntegerOverflow=off
  Product : Product
  Sign : Signum
  cyl_fric_up_to_100mm/s : Lookup_n-D  NumberOfTableDimensions=1  BreakpointsForDimension1=|  Table=|  InternalRulePriority=Speed  RndMeth=Simplest
      BreakpointsForDimension1=|
      | [0
      | 5
      | 10
      | 15
      | 20
      | 25
      | 30
      | 35
      | 40
      | 45
      | 50
      | 55
      | 60
      | 65
      | 70
      | 75
      | 80
      | 85
      | 90
      | 95
      | 100]./1e3;
      Table=|
      | [0
      | 242
      | 550
      | 838
      | 996
      | 972
      | 850
      | 757
      | 728
      | 733
      | 744
      | 753
      | 759
      | 765
      | 770
      | 775
      | 780
      | 785
      | 790
      | 795
      | 800];
  F_fric : Outport  VectorParamsAs1DForOutWhenUnconnected=off
  wires:
  Abs/1 -> cyl_fric_up_to_100mm/s/1
  v/1 -> Sign/1, Abs/1
  cyl_fric_up_to_100mm/s/1 -> Product/1
  Sign/1 -> Product/2
  Product/1 -> F_fric/1

== system copia 15_10_26/PLANTA/Actuador_Hidraulico_1/cylinder_63_36/volume A chamber ==
  note: ∆𝑉 = −𝑉0 / 𝐵𝑛 ∗ ∆𝑝
  Q_in : Inport
  " dV/dt" : Inport  Port=2
  " V" : Inport  Port=3
  " B" : Inport  Port=4
  Integrator : Integrator  InitialCondition=cyl.p0A  AbsoluteTolerance=10
  Product : Product  Inputs=*/*  InputSameDT=on  SaturateOnIntegerOverflow=on  OutDataTypeStr=Inherit: Same as first input
  Saturation : Saturate  UpperLimit=inf  LowerLimit=-1e5
  Sum1 : Sum  Inputs=+-  InputSameDT=on  SaturateOnIntegerOverflow=on  OutDataTypeStr=Inherit: Same as first input
  p : Outport  VectorParamsAs1DForOutWhenUnconnected=off
  wires:
  Integrator/1 -> Saturation/1
  Product/1 -> Integrator/1
  Sum1/1 -> Product/1
  " B"/1 -> Product/3
  Saturation/1 -> p/1
  Q_in/1 -> Sum1/1
  " V"/1 -> Product/2
  " dV/dt"/1 -> Sum1/2

== system copia 15_10_26/PLANTA/Actuador_Hidraulico_1/cylinder_63_36/volume B chamber ==
  Q_in : Inport
  " dV/dt" : Inport  Port=2
  " V" : Inport  Port=3
  " B" : Inport  Port=4
  Integrator : Integrator  InitialCondition=cyl.p0B  AbsoluteTolerance=10
  Product : Product  Inputs=*/*  InputSameDT=on  SaturateOnIntegerOverflow=on  OutDataTypeStr=Inherit: Same as first input
  Saturation : Saturate  UpperLimit=inf  LowerLimit=-1e5
  Sum1 : Sum  Inputs=+-  InputSameDT=on  SaturateOnIntegerOverflow=on  OutDataTypeStr=Inherit: Same as first input
  p : Outport  VectorParamsAs1DForOutWhenUnconnected=off
  wires:
  " dV/dt"/1 -> Sum1/2
  " V"/1 -> Product/2
  Q_in/1 -> Sum1/1
  Saturation/1 -> p/1
  " B"/1 -> Product/3
  Sum1/1 -> Product/1
  Product/1 -> Integrator/1
  Integrator/1 -> Saturation/1

== system copia 15_10_26/PLANTA/Actuador_Hidraulico_1/gate_load_mass/load_fric ==
  v : Inport
  Gain1 : Gain  Gain=-1
  Product : Product  Inputs=4
  Sign : Signum
  coeff_fric : Constant  Value=0.7e5
  F_fric_load : Outport  VectorParamsAs1DForOutWhenUnconnected=off
  wires:
  Product/1 -> F_fric_load/1
  Sign/1 -> Gain1/1
  coeff_fric/1 -> Product/4
  Gain1/1 -> Product/1
  v/1 -> Product/2, Product/3, Sign/1

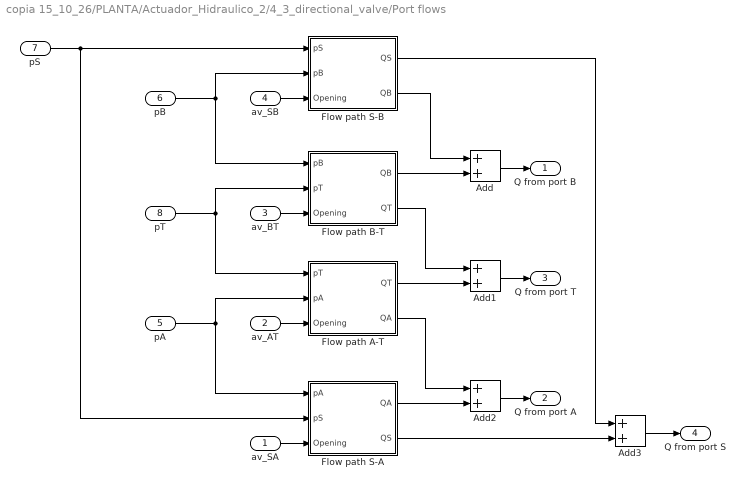
== system copia 15_10_26/PLANTA/Actuador_Hidraulico_2/4_3_directional_valve/Port flows ==
  av_SA : Inport
  av_AT : Inport  Port=2
  av_BT : Inport  Port=3
  av_SB : Inport  Port=4
  pA : Inport  Port=5
  pB : Inport  Port=6
  pS : Inport  Port=7
  pT : Inport  Port=8
  Add{,1..3} (4 alike) : Sum
  Flow path A-T : Subsystem  mask(Hydraulic){DPN=valve.dpN, QN=valve.QN, ptr=valve.ptr}
      mask prompts: DPN "Nominal Pressure Difference [Pa] :"; QN "Flow at nominal pressure difference and maximum opening [m^3/s] :"; ptr "Transition pressure [Pa] :"
      mask help:
      | Implements numerically robust turbulent flow equation. Polynomial flow equation is
      | used when abs(dp) is smaller than transition pressure.
      | [Source: Ellman, A. & Piche, R. 1996.
      | A Modified Orifice Flow Formula for Numerical Simulation of Fluid Power Systems.
      | Fluid Power Systems and Technology, ASME]
      mask init:
      | K = QN/(sqrt(DPN));
  Flow path B-T : Subsystem  mask(Hydraulic){DPN=valve.dpN, QN=valve.QN, ptr=valve.ptr}
      mask prompts: DPN "Nominal Pressure Difference [Pa] :"; QN "Flow at nominal pressure difference and maximum opening [m^3/s] :"; ptr "Transition pressure [Pa] :"
      mask help:
      | Implements numerically robust turbulent flow equation. Polynomial flow equation is
      | used when abs(dp) is smaller than transition pressure.
      | [Source: Ellman, A. & Piche, R. 1996.
      | A Modified Orifice Flow Formula for Numerical Simulation of Fluid Power Systems.
      | Fluid Power Systems and Technology, ASME]
      mask init:
      | K = QN/(sqrt(DPN));
  Flow path S-A : Subsystem  mask(Hydraulic){DPN=valve.dpN, QN=valve.QN, ptr=valve.ptr}
      mask prompts: DPN "Nominal Pressure Difference [Pa] :"; QN "Flow at nominal pressure difference and maximum opening [m^3/s] :"; ptr "Transition pressure [Pa] :"
      mask help:
      | Implements numerically robust turbulent flow equation. Polynomial flow equation is
      | used when abs(dp) is smaller than transition pressure.
      | [Source: Ellman, A. & Piche, R. 1996.
      | A Modified Orifice Flow Formula for Numerical Simulation of Fluid Power Systems.
      | Fluid Power Systems and Technology, ASME]
      mask init:
      | K = QN/(sqrt(DPN));
  Flow path S-B : Subsystem  mask(Hydraulic){DPN=valve.dpN, QN=valve.QN, ptr=valve.ptr}
      mask prompts: DPN "Nominal Pressure Difference [Pa] :"; QN "Flow at nominal pressure difference and maximum opening [m^3/s] :"; ptr "Transition pressure [Pa] :"
      mask help:
      | Implements numerically robust turbulent flow equation. Polynomial flow equation is
      | used when abs(dp) is smaller than transition pressure.
      | [Source: Ellman, A. & Piche, R. 1996.
      | A Modified Orifice Flow Formula for Numerical Simulation of Fluid Power Systems.
      | Fluid Power Systems and Technology, ASME]
      mask init:
      | K = QN/(sqrt(DPN));
  Q from port B : Outport  VectorParamsAs1DForOutWhenUnconnected=off
  Q from port A : Outport  Port=2  VectorParamsAs1DForOutWhenUnconnected=off
  Q from port T : Outport  Port=3  VectorParamsAs1DForOutWhenUnconnected=off
  Q from port S : Outport  Port=4  VectorParamsAs1DForOutWhenUnconnected=off
  wires:
  av_SA/1 -> Flow path S-A/3(Opening)
  av_AT/1 -> Flow path A-T/3(Opening)
  av_BT/1 -> Flow path B-T/3(Opening)
  pA/1 -> Flow path A-T/2(pA), Flow path S-A/1(pA)
  pB/1 -> Flow path B-T/1(pB), Flow path S-B/2(pB)
  pS/1 -> Flow path S-B/1(pS), Flow path S-A/2(pS)
  pT/1 -> Flow path A-T/1(pT), Flow path B-T/2(pT)
  Add/1 -> Q from port B/1
  Add1/1 -> Q from port T/1
  Add2/1 -> Q from port A/1
  Add3/1 -> Q from port S/1
  Flow path S-B/1(QS) -> Add3/1
  Flow path S-A/2(QS) -> Add3/2
  Flow path S-A/1(QA) -> Add2/2
  Flow path A-T/2(QA) -> Add2/1
  Flow path A-T/1(QT) -> Add1/2
  Flow path B-T/2(QT) -> Add1/1
  Flow path B-T/1(QB) -> Add/2
  Flow path S-B/2(QB) -> Add/1
  av_SB/1 -> Flow path S-B/3(Opening)

== system copia 15_10_26/PLANTA/Actuador_Hidraulico_2/4_3_directional_valve/Relative opening of flow paths ==
  x : Inport
  Gain : Gain  Gain=-1
  Lookup Table5 : Lookup  InputValues=[0.01 0.05 0.1 0.2 0.3 0.4 1]  Table=[0.01 0.039 0.078 0.16 0.23 0.31 0.78]  SaturateOnIntegerOverflow=off
  Lookup Table6 : Lookup  InputValues=[0.01 0.05 0.1 0.2 0.3 0.4 1]  Table=[0.01 0.036 0.072 0.14 0.22 0.29 0.72]  SaturateOnIntegerOverflow=off
  Lookup Table7 : Lookup  InputValues=[0.01 0.05 0.1 0.2 0.3 0.4 1]  Table=[0.01 0.039 0.077 0.15 0.23 0.31 0.77]  SaturateOnIntegerOverflow=off
  Lookup Table8 : Lookup  InputValues=[0.01 0.05 0.1 0.2 0.3 0.4 1]  Table=[0.01 0.035 0.070 0.14 0.21 0.28 0.70]  SaturateOnIntegerOverflow=off
  Saturation1 : Saturate  UpperLimit=1  LowerLimit=0
  Saturation2 : Saturate  UpperLimit=0  LowerLimit=-1
  av_SA : Outport  VectorParamsAs1DForOutWhenUnconnected=off
  av_AT : Outport  Port=2  VectorParamsAs1DForOutWhenUnconnected=off
  av_BT : Outport  Port=3  VectorParamsAs1DForOutWhenUnconnected=off
  av_SB : Outport  Port=4  VectorParamsAs1DForOutWhenUnconnected=off
  wires:
  x/1 -> Saturation2/1, Saturation1/1
  Saturation2/1 -> Gain/1
  Lookup Table8/1 -> av_AT/1
  Lookup Table7/1 -> av_SB/1
  Lookup Table6/1 -> av_BT/1
  Lookup Table5/1 -> av_SA/1
  Saturation1/1 -> Lookup Table5/1, Lookup Table6/1
  Gain/1 -> Lookup Table8/1, Lookup Table7/1

== system copia 15_10_26/PLANTA/Actuador_Hidraulico_2/4_3_directional_valve/Valve dynamics ==
  u : Inport
  Rate Limiter : RateLimiter  RisingSlewLimit=valve.ratelimit  FallingSlewLimit=-valve.ratelimit  SampleTimeMode=inherited
  Saturation limits [-1,1] : Saturate  UpperLimit=1  LowerLimit=-1
  Saturation limits [-1,1]2 : Saturate  UpperLimit=1  LowerLimit=-1
  Transfer Fcn1 : TransferFcn  Denominator=[valve.tau 1]
  Transport Delay of the valve : TransportDelay  DelayTime=valve.delay
  x : Outport  VectorParamsAs1DForOutWhenUnconnected=off
  wires:
  Saturation limits [-1,1]/1 -> Transport Delay of the valve/1
  Transport Delay of the valve/1 -> Rate Limiter/1
  Rate Limiter/1 -> Transfer Fcn1/1
  u/1 -> Saturation limits [-1,1]/1
  Transfer Fcn1/1 -> Saturation limits [-1,1]2/1
  Saturation limits [-1,1]2/1 -> x/1

== system copia 15_10_26/PLANTA/Actuador_Hidraulico_2/cylinder_63_36/A-chamber and pipe size submodel ==
  x_cyl : Inport
  A : Gain  Gain=pipe.area
  A chamber dead volume : Constant  Value=cyl.V0A
  Add : Sum  Inputs=+++
  Gain : Gain  Gain=cyl.A_piston
  Lenght : Constant  Value=pipe.lenght
  V : Outport  VectorParamsAs1DForOutWhenUnconnected=off
  wires:
  A/1 -> Add/3
  Lenght/1 -> A/1
  A chamber dead volume/1 -> Add/2
  Gain/1 -> Add/1
  x_cyl/1 -> Gain/1
  Add/1 -> V/1

== system copia 15_10_26/PLANTA/Actuador_Hidraulico_2/cylinder_63_36/B-chamber and pipe size submodel ==
  x_cyl : Inport
  A : Gain  Gain=pipe.area
  Add : Sum  Inputs=+-
  Add1 : Sum  Inputs=+++
  B chamber dead volume : Constant  Value=cyl.V0B
  Cylinder stroke : Constant  Value=cyl.stroke
  Gain1 : Gain  Gain=cyl.A_rodside
  Lenght : Constant  Value=pipe.lenght
  V : Outport  VectorParamsAs1DForOutWhenUnconnected=off
  wires:
  A/1 -> Add1/3
  Lenght/1 -> A/1
  Cylinder stroke/1 -> Add/1
  Gain1/1 -> Add1/1
  Add/1 -> Gain1/1
  x_cyl/1 -> Add/2
  B chamber dead volume/1 -> Add1/2
  Add1/1 -> V/1

== system copia 15_10_26/PLANTA/Actuador_Hidraulico_2/cylinder_63_36/dynamic_fric_limited ==
  v : Inport
  Abs : Abs  SaturateOnIntegerOverflow=off
  Product : Product
  Sign : Signum
  cyl_fric_up_to_100mm/s : Lookup_n-D  NumberOfTableDimensions=1  BreakpointsForDimension1=|  Table=|  InternalRulePriority=Speed  RndMeth=Simplest
      BreakpointsForDimension1=|
      | [0
      | 5
      | 10
      | 15
      | 20
      | 25
      | 30
      | 35
      | 40
      | 45
      | 50
      | 55
      | 60
      | 65
      | 70
      | 75
      | 80
      | 85
      | 90
      | 95
      | 100]./1e3;
      Table=|
      | [0
      | 242
      | 550
      | 838
      | 996
      | 972
      | 850
      | 757
      | 728
      | 733
      | 744
      | 753
      | 759
      | 765
      | 770
      | 775
      | 780
      | 785
      | 790
      | 795
      | 800];
  F_fric : Outport  VectorParamsAs1DForOutWhenUnconnected=off
  wires:
  Abs/1 -> cyl_fric_up_to_100mm/s/1
  v/1 -> Sign/1, Abs/1
  cyl_fric_up_to_100mm/s/1 -> Product/1
  Sign/1 -> Product/2
  Product/1 -> F_fric/1
